simulink model "microgrid_top"  (R2025a)
settings: Solver=FixedStepDiscrete  StartTime=0.0  StopTime=86400  FixedStep=Ts  RelTol=1e-3
InitFcn:
  | init_microgrid
undefined symbols (not defined in the file): d, dt, Emax, G_clear_day, Ion, Lithium, Pmax, prof, sig, SoC_min, T_amb_day, t_day, t_hour, Tc, th1, th1_act, th2, th2_act, Ts
libraries: spsSeriesRLCBranchLib x9, spsMosfetLib x8, simulink x7, spsIGBTDiodeLib x4, slpidlib x4, spsIdealSwitchLib x4, spsVoltageMeasurementLib x4, spsParallelRLCLoadLib x3, spsPWMGeneratorDCDCLib x2, spsCurrentMeasurementLib x2, spsBatteryLib x1, spsFirstOrderFilterLib x1
settings Model: Creator=mdnih  LastModifiedBy=mdnih
settings SolverCC: AutoInsertRateTranBlk=on

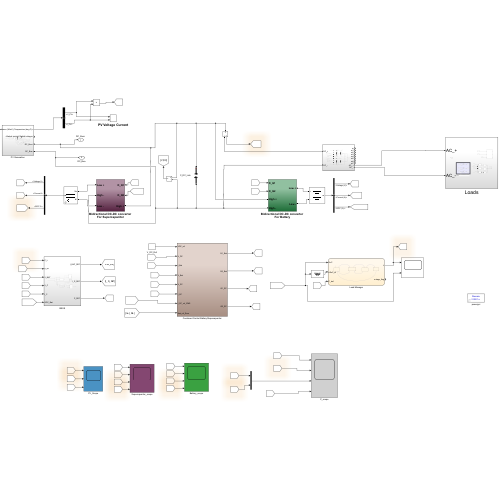
[thumbnail: Simulink's stored preview of the top-level diagram]
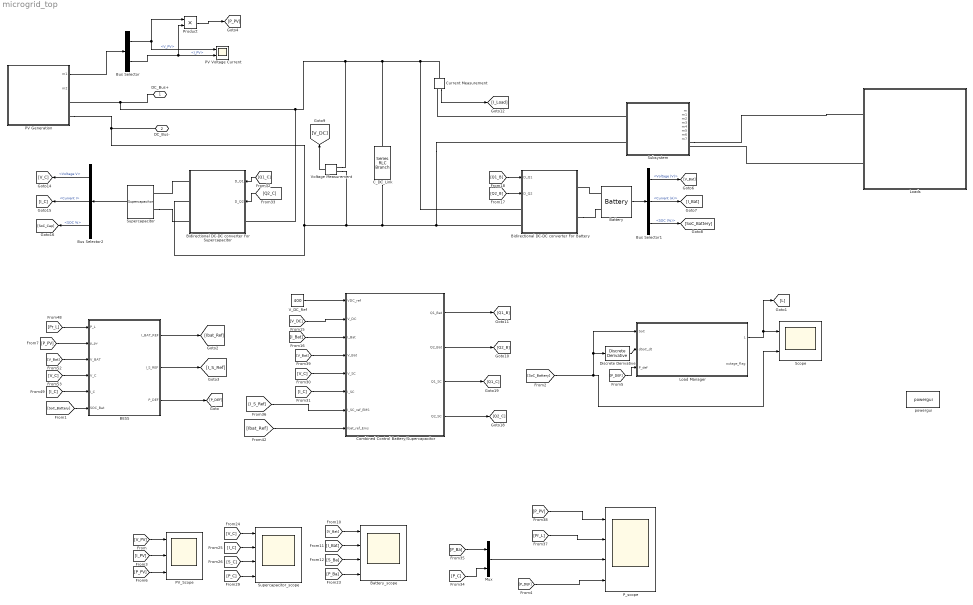
== system microgrid_top ==
  BESS : Subsystem
  Battery : spsBatteryLib/Battery  BatType=Lithium-Ion  NomV=24  NomQ=14  SOC=50  Batt_Tr=0.1  PresetModel=on  MaxQ=14  MinV=18  FullV=27.9357  Dis_rate=6.087  R=0.017143  Normal_OP=12.6609  expZone="[25.9293     0.687826]"
      settings: LibrarySourceBlock=electricdrivelib/Extra Sources/Battery
  "Battery_scope " : Scope  NumInputPorts=4
      settings: ActiveDisplayYMinimum=-3.2401785596786041  ActiveDisplayYMaximum=29.161607037107444  DataLoggingVariableName=ScopeData2
  Bidirectional DC-DC converter For Battery : Subsystem
  Bidirectional DC-DC converter For Supercapacitor : Subsystem
  Bus Selector : BusSelector  OutputSignals=V_PV,I_PV
  Bus Selector1 : BusSelector  OutputSignals=Voltage (V),Current (A),SOC (%)
  Bus Selector2 : BusSelector  OutputSignals=Voltage V,Current I,SOC %
  C_DC_Link : spsSeriesRLCBranchLib/Series RLC Branch  LConnTagsString=__new0  RConnTagsString=__new0  BranchType=C  Resistance=1  Inductance=1e-3  SetiL0=off  InitialCurrent=0  Capacitance=300e-6  Setx0=off  InitialVoltage=0  Measurements=None
  Combined Control Battery/Supercapacitor : Subsystem
  Current Measurement : spsCurrentMeasurementLib/Current Measurement  PhasorSimulation=off  OutputType=Complex  PSBequivalent=0
  Discrete Derivative : simulink/Discrete/Discrete Derivative  gainval=1.0  ICPrevScaledInput=0.0  OutMin=[]  OutMax=[]  OutDataType=fixdt(1, 16)  OutScaling=2^-10  DoSatur=off
  Load Manager : Stateflow chart  TreatAsAtomicUnit=on
  Loads : Subsystem
  Mux : Mux  Inputs=2
  PV Generation : Subsystem
  PV Voltage Current : Scope  NumInputPorts=2
  PV_Scope : Scope  NumInputPorts=3
      settings: ActiveDisplayYMinimum=-5.01178  ActiveDisplayYMaximum=45.10602  DataLoggingVariableName=ScopeData3
  P_scope : Scope  NumInputPorts=4
      settings: ActiveDisplayYMinimum=-1  ActiveDisplayYMaximum=1  DataLoggingVariableName=ScopeData4
  Product : Product
  Scope : Scope  NumInputPorts=2
      settings: ActiveDisplayYMinimum=-0.24999999999999994  ActiveDisplayYMaximum=2.25
  Subsystem : Subsystem
  Supercapacitor : spsSupercapacitorLib/Supercapacitor  C=29  Rdc=0.003  Voltage=32  Ns=1  Np=1  Vinit=32  Temp=25  Nc=1  r=1e-9  epsilon=6.0208e-10  Ioc=10  Vself="[48  47.8  47.06  44.65]"
      settings: LibrarySourceBlock=electricdrivelib/Extra Sources/Supercapacitor
  Supercapacitor_scope : Scope  NumInputPorts=4
      settings: ActiveDisplayYMinimum=31.852425698954992  ActiveDisplayYMaximum=32.0163550827263  DataLoggingVariableName=ScopeData5
  V_DC_Ref : Constant  Value=400
  Voltage Measurement : spsVoltageMeasurementLib/Voltage Measurement  PhasorSimulation=off  OutputType=Complex  PSBequivalent=0
  powergui : sps_lib/powergui  Priority=1  SimulationMode=Discrete  SampleTime=Ts  frequency=60  Iterations=50  frequencyindice=0  Pbase=100e6  ErrMax=1e-4  UnitsV=kV  UnitsW=MW  buscounter=0  FunctionMessages=off  echomessages=off  EnableUseOfTLC=off  CurrentSourceSwitches=off  DisableSnubberDevices=off  DisableRonSwitches=off  DisableVfSwitches=off  DisplayEquations=off  AutomaticDiscreteSolvers=off  SolverType=Tustin/Backward Euler (TBE)  Interpol=off  ExternalGateDelay=off  methode=off  Ts=100  x0status=blocks  SPID=on  SwTol=0  HookPort=off  NonlinearTolerance=1e-4  nMaxIteration=100  ContinueOnMaxIteration=off  RestoreLinks=warning  ResistiveCurrentMeasurement=off  Frange=[0:2:500]  Ylog=off  Xlog=on  ShowGrid=off  save=off  variable=ZData  structure=0  ZoomFFT=off  StartTime=0.0  cycles=1  DisplayStyle=1  fundamental=60  FreqAxis=off  MaxFrequency=1000  frequencyindicesteady=1  RmsSteady=1  display=off
  DC_Bus+ : PMIOPort  Side=Right
  DC_Bus- : PMIOPort  Port=2  Side=Left
  wires:
  [Q1_B] -> Bidirectional DC-DC converter For Battery/1(D_Q1)
  Bus Selector2/1 -> [V_C]  "<Voltage V>"
  [Q2_B] -> Bidirectional DC-DC converter For Battery/2(D_Q2)
  Battery/1 -> Bus Selector1/1
  Bus Selector1/3 -> [SoC_Battery]  "<SOC (%)>"
  Bus Selector1/2 -> [I_Bat]  "<Current (A)>"
  Voltage Measurement/1 -> [V_DC]
  Bus Selector1/1 -> [V_Bat]  "<Voltage (V)>"
  [Q2_C] -> Bidirectional DC-DC converter For Supercapacitor/2(D_Q2)
  Bus Selector2/2 -> [I_C]  "<Current I>"
  Supercapacitor/1 -> Bus Selector2/1
  Current Measurement/1 -> [I_Load]
  Bus Selector2/3 -> [SoC_Cap]  "<SOC %>"
  [Q1_C] -> Bidirectional DC-DC converter For Supercapacitor/1(D_Q1)
  [SoC_Battery] -> BESS/6(SOC_Bat)
  [Pr_L] -> BESS/1(P_L)
  [V_C] -> BESS/4(V_C)
  [P_PV] -> BESS/2(p_pv)
  [V_Bat] -> BESS/3(V_BAT)
  BESS/2(I_S_REF) -> [I_S_Ref]
  BESS/3(P_DEF) -> [P_DEF]
  BESS/1(I_BAT_REF) -> [Ibat_Ref]
  [I_C] -> BESS/5(I_C)
  [SoC_Battery] -> Scope/2, Discrete Derivative/1, Load Manager/1(SoC)
  PV Generation/1(m1) -> Bus Selector/1
  Bus Selector/1 -> Product/1, PV Voltage Current/1  "<V_PV>"
  Bus Selector/2 -> Product/2, PV Voltage Current/2  "<I_PV>"
  [I_S_Ref] -> Combined Control Battery/Supercapacitor/7(I_SC_ref_EMS)
  [V_Bat] -> Combined Control Battery/Supercapacitor/4(V_Bat)
  Combined Control Battery/Supercapacitor/3(Q1_SC) -> [Q1_C]
  Combined Control Battery/Supercapacitor/4(Q2_SC) -> [Q2_C]
  [V_C] -> Combined Control Battery/Supercapacitor/5("V_SC ")
  Combined Control Battery/Supercapacitor/2(Q2_Bat) -> [Q2_B]
  [I_Bat] -> Combined Control Battery/Supercapacitor/3(I_Bat)
  Combined Control Battery/Supercapacitor/1(Q1_Bat) -> [Q1_B]
  [I_C] -> Combined Control Battery/Supercapacitor/6(I_SC)
  [Ibat_Ref] -> Combined Control Battery/Supercapacitor/8(Ibat_ref_Ems)
  [V_DC] -> Combined Control Battery/Supercapacitor/2(V_DC)
  V_DC_Ref/1 -> Combined Control Battery/Supercapacitor/1(VDC_ref)
  [P_Ba] -> "Battery_scope "/4
  [P_Ba] -> Mux/1
  [Pr_L] -> P_scope/2
  [V_PV] -> PV_Scope/1
  [P_C] -> Mux/2
  [P_DEF] -> P_scope/4
  [S_C] -> Supercapacitor_scope/3
  [V_C] -> Supercapacitor_scope/1
  [I_Bat] -> "Battery_scope "/2
  [P_PV] -> P_scope/1
  [P_PV] -> PV_Scope/3
  [S_Ba] -> "Battery_scope "/3
  Mux/1 -> P_scope/3
  [P_C] -> Supercapacitor_scope/4
  [V_Bat] -> "Battery_scope "/1
  [I_C] -> Supercapacitor_scope/2
  [I_PV] -> PV_Scope/2
  Load Manager/1(L) -> [L], Scope/1
  Discrete Derivative/1 -> Load Manager/2(dSoC_dt)
  [P_DEF] -> Load Manager/3(P_def)
  Product/1 -> [P_PV]
  connections:
  PV Generation/RConn2 -- DC_Bus-/RConn1 -- Voltage Measurement/LConn2 -- Subsystem/LConn2 -- Bidirectional DC-DC converter For Battery/LConn2 -- C_DC_Link/RConn1 -- Bidirectional DC-DC converter For Supercapacitor/RConn2
  DC_Bus+/RConn1 -- PV Generation/RConn1 -- Voltage Measurement/LConn1 -- Current Measurement/LConn1 -- Bidirectional DC-DC converter For Battery/LConn1 -- C_DC_Link/LConn1 -- Bidirectional DC-DC converter For Supercapacitor/LConn1
  Subsystem/LConn1 -- Current Measurement/RConn1
  Supercapacitor/LConn2 -- Bidirectional DC-DC converter For Supercapacitor/RConn3
  Bidirectional DC-DC converter For Supercapacitor/RConn1 -- Supercapacitor/LConn1
  Battery/LConn1 -- Bidirectional DC-DC converter For Battery/RConn1
  Bidirectional DC-DC converter For Battery/RConn2 -- Battery/LConn2
  Subsystem/RConn1 -- Loads/LConn1
  Loads/LConn2 -- Subsystem/RConn2

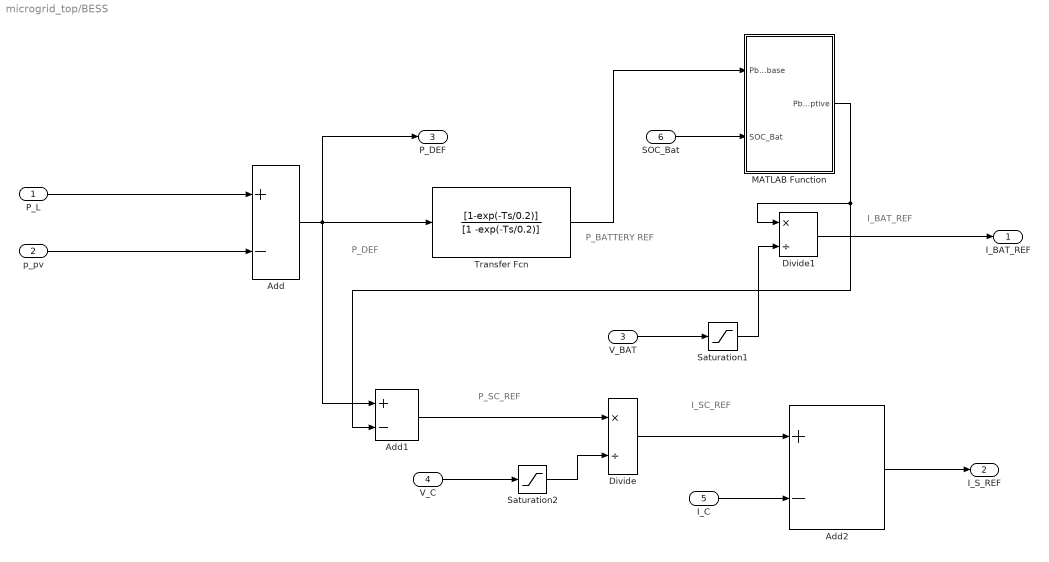
== system microgrid_top/BESS ==
  note: P_SC_REF
  note: I_BAT_REF
  note: P_DEF
  note: P_BATTERY REF
  note: I_SC_REF
  P_L : Inport
  p_pv : Inport  Port=2
  V_BAT : Inport  Port=3
  V_C : Inport  Port=4
  I_C : Inport  Port=5
  SOC_Bat : Inport  Port=6
  Add : Sum  Inputs=+-
  Add1 : Sum  Inputs=+-
  Add2 : Sum  Inputs=+-
  Divide : Product  Inputs=*/
  Divide1 : Product  Inputs=*/
  MATLAB Function : MATLAB Function  TreatAsAtomicUnit=on
  Saturation1 : Saturate  UpperLimit=1000  LowerLimit=1
  Saturation2 : Saturate  UpperLimit=1000  LowerLimit=1
  Transfer Fcn : DiscreteTransferFcn  Numerator=[1-exp(-Ts/0.2)]  Denominator=[1 -exp(-Ts/0.2)]  SampleTime=Ts
  I_BAT_REF : Outport
  I_S_REF : Outport  Port=2
  P_DEF : Outport  Port=3
  wires:
  Transfer Fcn/1 -> MATLAB Function/1(Pbat_base)
  Add1/1 -> Divide/1
  Saturation2/1 -> Divide/2
  MATLAB Function/1(Pbat_adaptive) -> Add1/2, Divide1/1
  Add/1 -> P_DEF/1, Transfer Fcn/1, Add1/1
  Saturation1/1 -> Divide1/2
  Divide/1 -> Add2/1
  P_L/1 -> Add/1
  p_pv/1 -> Add/2
  SOC_Bat/1 -> MATLAB Function/2(SOC_Bat)
  Divide1/1 -> I_BAT_REF/1
  Add2/1 -> I_S_REF/1
  V_BAT/1 -> Saturation1/1
  I_C/1 -> Add2/2
  V_C/1 -> Saturation2/1

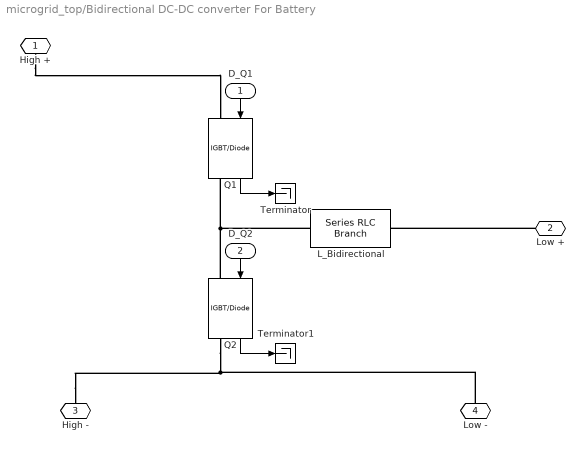
== system microgrid_top/Bidirectional DC-DC converter For Battery ==
  D_Q1 : Inport
  D_Q2 : Inport  Port=2
  L_Bidirectional : spsSeriesRLCBranchLib/Series RLC Branch  LConnTagsString=__new0  RConnTagsString=__new0  BranchType=RL  Resistance=0.05  Inductance=0.3e-3  SetiL0=off  InitialCurrent=0  Capacitance=1e-6  Setx0=off  InitialVoltage=0  Measurements=None
  Q1 : spsIGBTDiodeLib/IGBT//Diode  Ron=1e-3  Rs=1e5  Cs=inf  Measurements=on
  Q2 : spsIGBTDiodeLib/IGBT//Diode  Ron=1e-3  Rs=1e5  Cs=inf  Measurements=on
  Terminator : Terminator
  Terminator1 : Terminator
  High + : PMIOPort  Side=Left
  Low + : PMIOPort  Port=2  Side=Right
  High - : PMIOPort  Port=3  Side=Left
  Low - : PMIOPort  Port=4  Side=Right
  wires:
  D_Q2/1 -> Q2/1
  D_Q1/1 -> Q1/1
  Q1/1 -> Terminator/1
  Q2/1 -> Terminator1/1
  connections:
  High -/RConn1 -- Low -/RConn1 -- Q2/RConn1
  High +/RConn1 -- Q1/LConn1
  Low +/RConn1 -- L_Bidirectional/RConn1
  Q2/LConn1 -- L_Bidirectional/LConn1 -- Q1/RConn1

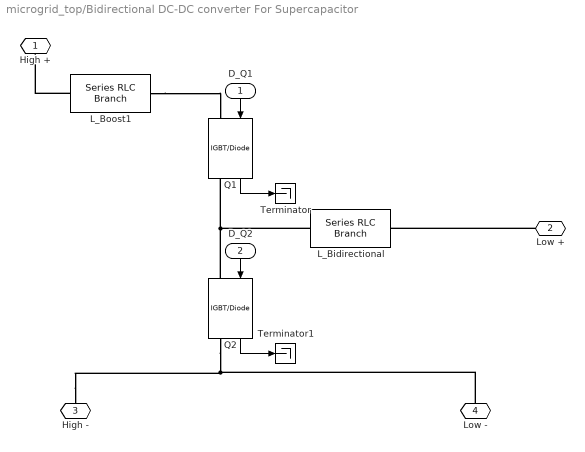
== system microgrid_top/Bidirectional DC-DC converter For Supercapacitor ==
  D_Q1 : Inport
  D_Q2 : Inport  Port=2
  L_Bidirectional : spsSeriesRLCBranchLib/Series RLC Branch  LConnTagsString=__new0  RConnTagsString=__new0  BranchType=RL  Resistance=0.05  Inductance=0.355e-3  SetiL0=off  InitialCurrent=0  Capacitance=1e-6  Setx0=off  InitialVoltage=0  Measurements=None
  L_Boost1 : spsSeriesRLCBranchLib/Series RLC Branch  LConnTagsString=__new0  RConnTagsString=__new0  BranchType=L  Resistance=0.05  Inductance=1.5e-3  SetiL0=off  InitialCurrent=0  Capacitance=1e-6  Setx0=off  InitialVoltage=0  Measurements=None
  Q1 : spsIGBTDiodeLib/IGBT//Diode  Ron=1e-3  Rs=1e5  Cs=inf  Measurements=on
  Q2 : spsIGBTDiodeLib/IGBT//Diode  Ron=1e-3  Rs=1e5  Cs=inf  Measurements=on
  Terminator : Terminator
  Terminator1 : Terminator
  High + : PMIOPort  Side=Left
  Low + : PMIOPort  Port=2  Side=Right
  High - : PMIOPort  Port=3  Side=Right
  Low - : PMIOPort  Port=4  Side=Right
  wires:
  D_Q2/1 -> Q2/1
  D_Q1/1 -> Q1/1
  Q1/1 -> Terminator/1
  Q2/1 -> Terminator1/1
  connections:
  High -/RConn1 -- Low -/RConn1 -- Q2/RConn1
  Low +/RConn1 -- L_Bidirectional/RConn1
  Q2/LConn1 -- L_Bidirectional/LConn1 -- Q1/RConn1
  L_Boost1/RConn1 -- Q1/LConn1
  L_Boost1/LConn1 -- High +/RConn1

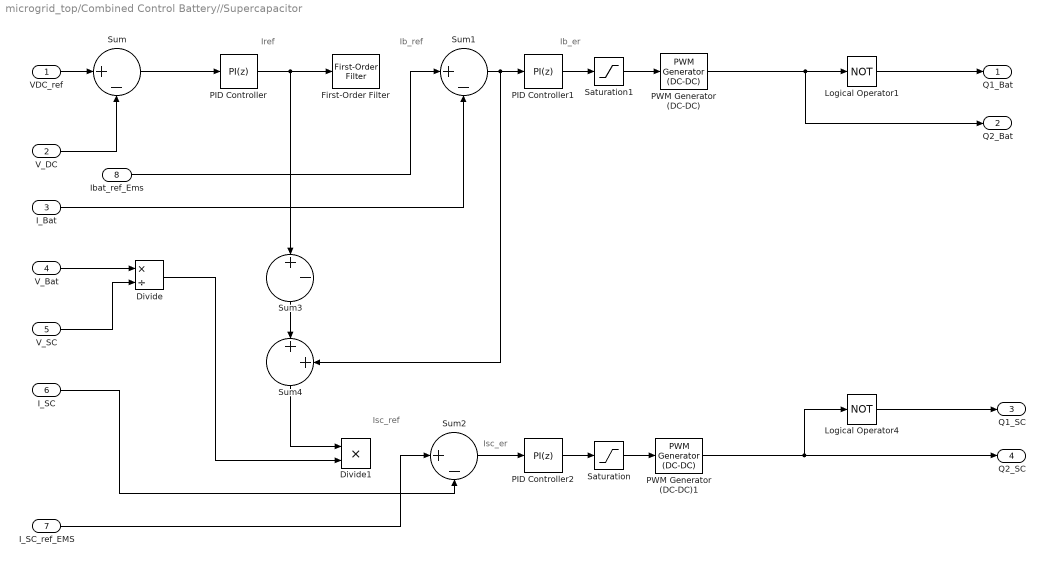
== system microgrid_top/Combined Control Battery//Supercapacitor ==
  note: Isc_er
  note: Isc_ref
  note: Ib_er
  note: Ib_ref
  note: Iref
  VDC_ref : Inport
  V_DC : Inport  Port=2
  I_Bat : Inport  Port=3
  V_Bat : Inport  Port=4
  "V_SC " : Inport  Port=5
  I_SC : Inport  Port=6
  I_SC_ref_EMS : Inport  Port=7
  Ibat_ref_Ems : Inport  Port=8
  Divide : Product  Inputs=*/
  Divide1 : Product  Inputs=**
  First-Order Filter : spsFirstOrderFilterLib/First-Order Filter  FilterType=Lowpass  Tc=0.015  Ts=Ts  Initialize=off  Vac_Init=[0, 0, 60]  Vdc_Init=0  PlotResponse=off  FreqRange="[0,  200,  1]"
  Logical Operator1 : Logic  Operator=NOT  AllPortsSameDT=off  OutDataTypeStr=boolean
  Logical Operator4 : Logic  Operator=NOT  AllPortsSameDT=off  OutDataTypeStr=boolean
  PID Controller : slpidlib/PID Controller  Controller=PI  Form=Parallel  TimeDomain=Discrete-time  UseExternalTs=off  SampleTime=Ts  IntegratorMethod=Backward Euler  FilterMethod=Backward Euler  ControllerParametersSource=internal  P=1.477  I=3077  UseKiTs=off  D=0  UseExternalDerivativeSource=off  N=100  UseFilter=on  TunerSelectOption=Transfer Function Based (PID Tuner App)  InitialConditionSource=internal  InitialConditionForIntegrator=0  InitialConditionForFilter=0  DifferentiatorICPrevScaledInput=0  ExternalReset=none  TrackingMode=off  Kt=1  LimitOutput=off  SatLimitsSource=internal  UpperSaturationLimit=inf  LowerSaturationLimit=-inf  LinearizeAsGain=on  AntiWindupMode=none  Kb=1  LimitIntegrator=off  UpperIntegratorSaturationLimit=inf  LowerIntegratorSaturationLimit=-inf  POutMin=[]  POutMax=[]  IOutMin=[]  IOutMax=[]  DOutMin=[]  DOutMax=[]  NOutMin=[]  NOutMax=[]  SumOutMin=[]  SumOutMax=[]  SaturationOutMin=[]  SaturationOutMax=[]  PParamMin=[]  PParamMax=[]  IParamMin=[]  IParamMax=[]  DParamMin=[]  DParamMax=[]  NParamMin=[]  NParamMax=[]  KbParamMin=[]  KbParamMax=[]  KtParamMin=[]  KtParamMax=[]  KbOutMin=[]  KbOutMax=[]  KtOutMin=[]  KtOutMax=[]  IntegratorOutMin=[]  IntegratorOutMax=[]  FilterOutMin=[]  FilterOutMax=[]  SumI1OutMin=[]  SumI1OutMax=[]  SumI2OutMin=[]  SumI2OutMax=[]  SumI3OutMin=[]  SumI3OutMax=[]  SumI4OutMin=[]  SumI4OutMax=[]  SumDOutMin=[]  SumDOutMax=[]  DifferentiatorOutMin=[]  DifferentiatorOutMax=[]  FilterDiffOutCoefMin=[]  FilterDiffOutCoefMax=[]  ReciprocalOutMin=[]  ReciprocalOutMax=[]  SumDenOutMin=[]  SumDenOutMax=[]  SumNumOutMin=[]  SumNumOutMax=[]  DivideOutMin=[]  DivideOutMax=[]  UdiffTsProdOutMin=[]  UdiffTsProdOutMax=[]  NTsProdOutMin=[]  NTsProdOutMax=[]  UintegralTsProdOutMin=[]  UintegralTsProdOutMax=[]  UngainTsProdOutMin=[]  UngainTsProdOutMax=[]  ClampingZeroOutDataTypeStr=Inherit: Inherit via back propagation  ClampingZeroOutMin=[]  ClampingZeroOutMax=[]  FilterDenConstantOutDataTypeStr=Inherit: Inherit via back propagation  FilterDenConstantOutMin=[]  FilterDenConstantOutMax=[]  PCopyOutDataTypeStr=Inherit: Inherit via back propagation  PCopyOutMin=[]  PCopyOutMax=[]  NCopyOutDataTypeStr=Inherit: Inherit via back propagation  NCopyOutMin=[]  NCopyOutMax=[]  IntegratorContinuousStateAttributes=''  IntegratorStateMustResolveToSignalObject=off  IntegratorRTWStateStorageClass=Auto  FilterContinuousStateAttributes=''  FilterStateMustResolveToSignalObject=off  FilterRTWStateStorageClass=Auto  ParallelPVariant=InternalParameters  IdealPVariant=Disabled  IVariant=InternalParameters  DVariant=Disabled  IntegratorVariant=Discrete  SatVariant=Disabled  AWVariant=Passthrough  PCopyVariant=Disabled  TRVariant=Disabled  FdbkBlocksVariant=Forward  IdealPFdbkVariant=Disabled  SatFdbkVariant=Disabled  DerivativeFilterVariant=Disabled  NVariant=Disabled  NCopyVariant=Disabled_SignalSpec  FilterICVariant=Disabled  IntegratorICVariant=InternalICs  ExternalResetVariant=Disabled  TRSumVariant=Passthrough  SumFdbkVariant=Disabled  SumVariant=Sum_PI  TsampFilterVariant=InternalTs  TsampNgainVariant=Passthrough  TsampIntegralVariant=Disabled_SignalSpec  ExternalSaturationOutDataTypeStr=Inherit: Same as second input  DerivativeSourceVariant=Disabled  PreIntVariant=InternalPreInt
  PID Controller1 : slpidlib/PID Controller  Controller=PI  Form=Parallel  TimeDomain=Discrete-time  UseExternalTs=off  SampleTime=Ts  IntegratorMethod=Backward Euler  FilterMethod=Backward Euler  ControllerParametersSource=internal  P=0.043  I=0.65  UseKiTs=off  D=0  UseExternalDerivativeSource=off  N=100  UseFilter=on  TunerSelectOption=Transfer Function Based (PID Tuner App)  InitialConditionSource=internal  InitialConditionForIntegrator=0  InitialConditionForFilter=0  DifferentiatorICPrevScaledInput=0  ExternalReset=none  TrackingMode=off  Kt=1  LimitOutput=off  SatLimitsSource=internal  UpperSaturationLimit=inf  LowerSaturationLimit=-inf  LinearizeAsGain=on  AntiWindupMode=none  Kb=1  LimitIntegrator=off  UpperIntegratorSaturationLimit=inf  LowerIntegratorSaturationLimit=-inf  POutMin=[]  POutMax=[]  IOutMin=[]  IOutMax=[]  DOutMin=[]  DOutMax=[]  NOutMin=[]  NOutMax=[]  SumOutMin=[]  SumOutMax=[]  SaturationOutMin=[]  SaturationOutMax=[]  PParamMin=[]  PParamMax=[]  IParamMin=[]  IParamMax=[]  DParamMin=[]  DParamMax=[]  NParamMin=[]  NParamMax=[]  KbParamMin=[]  KbParamMax=[]  KtParamMin=[]  KtParamMax=[]  KbOutMin=[]  KbOutMax=[]  KtOutMin=[]  KtOutMax=[]  IntegratorOutMin=[]  IntegratorOutMax=[]  FilterOutMin=[]  FilterOutMax=[]  SumI1OutMin=[]  SumI1OutMax=[]  SumI2OutMin=[]  SumI2OutMax=[]  SumI3OutMin=[]  SumI3OutMax=[]  SumI4OutMin=[]  SumI4OutMax=[]  SumDOutMin=[]  SumDOutMax=[]  DifferentiatorOutMin=[]  DifferentiatorOutMax=[]  FilterDiffOutCoefMin=[]  FilterDiffOutCoefMax=[]  ReciprocalOutMin=[]  ReciprocalOutMax=[]  SumDenOutMin=[]  SumDenOutMax=[]  SumNumOutMin=[]  SumNumOutMax=[]  DivideOutMin=[]  DivideOutMax=[]  UdiffTsProdOutMin=[]  UdiffTsProdOutMax=[]  NTsProdOutMin=[]  NTsProdOutMax=[]  UintegralTsProdOutMin=[]  UintegralTsProdOutMax=[]  UngainTsProdOutMin=[]  UngainTsProdOutMax=[]  ClampingZeroOutDataTypeStr=Inherit: Inherit via back propagation  ClampingZeroOutMin=[]  ClampingZeroOutMax=[]  FilterDenConstantOutDataTypeStr=Inherit: Inherit via back propagation  FilterDenConstantOutMin=[]  FilterDenConstantOutMax=[]  PCopyOutDataTypeStr=Inherit: Inherit via back propagation  PCopyOutMin=[]  PCopyOutMax=[]  NCopyOutDataTypeStr=Inherit: Inherit via back propagation  NCopyOutMin=[]  NCopyOutMax=[]  IntegratorContinuousStateAttributes=''  IntegratorStateMustResolveToSignalObject=off  IntegratorRTWStateStorageClass=Auto  FilterContinuousStateAttributes=''  FilterStateMustResolveToSignalObject=off  FilterRTWStateStorageClass=Auto  ParallelPVariant=InternalParameters  IdealPVariant=Disabled  IVariant=InternalParameters  DVariant=Disabled  IntegratorVariant=Discrete  SatVariant=Disabled  AWVariant=Passthrough  PCopyVariant=Disabled  TRVariant=Disabled  FdbkBlocksVariant=Forward  IdealPFdbkVariant=Disabled  SatFdbkVariant=Disabled  DerivativeFilterVariant=Disabled  NVariant=Disabled  NCopyVariant=Disabled_SignalSpec  FilterICVariant=Disabled  IntegratorICVariant=InternalICs  ExternalResetVariant=Disabled  TRSumVariant=Passthrough  SumFdbkVariant=Disabled  SumVariant=Sum_PI  TsampFilterVariant=InternalTs  TsampNgainVariant=Passthrough  TsampIntegralVariant=Disabled_SignalSpec  ExternalSaturationOutDataTypeStr=Inherit: Same as second input  DerivativeSourceVariant=Disabled  PreIntVariant=InternalPreInt
  PID Controller2 : slpidlib/PID Controller  Controller=PI  Form=Parallel  TimeDomain=Discrete-time  UseExternalTs=off  SampleTime=Ts  IntegratorMethod=Backward Euler  FilterMethod=Backward Euler  ControllerParametersSource=internal  P=0.45  I=14800  UseKiTs=off  D=0  UseExternalDerivativeSource=off  N=100  UseFilter=on  TunerSelectOption=Transfer Function Based (PID Tuner App)  InitialConditionSource=internal  InitialConditionForIntegrator=0  InitialConditionForFilter=0  DifferentiatorICPrevScaledInput=0  ExternalReset=none  TrackingMode=off  Kt=1  LimitOutput=off  SatLimitsSource=internal  UpperSaturationLimit=inf  LowerSaturationLimit=-inf  LinearizeAsGain=on  AntiWindupMode=none  Kb=1  LimitIntegrator=off  UpperIntegratorSaturationLimit=inf  LowerIntegratorSaturationLimit=-inf  POutMin=[]  POutMax=[]  IOutMin=[]  IOutMax=[]  DOutMin=[]  DOutMax=[]  NOutMin=[]  NOutMax=[]  SumOutMin=[]  SumOutMax=[]  SaturationOutMin=[]  SaturationOutMax=[]  PParamMin=[]  PParamMax=[]  IParamMin=[]  IParamMax=[]  DParamMin=[]  DParamMax=[]  NParamMin=[]  NParamMax=[]  KbParamMin=[]  KbParamMax=[]  KtParamMin=[]  KtParamMax=[]  KbOutMin=[]  KbOutMax=[]  KtOutMin=[]  KtOutMax=[]  IntegratorOutMin=[]  IntegratorOutMax=[]  FilterOutMin=[]  FilterOutMax=[]  SumI1OutMin=[]  SumI1OutMax=[]  SumI2OutMin=[]  SumI2OutMax=[]  SumI3OutMin=[]  SumI3OutMax=[]  SumI4OutMin=[]  SumI4OutMax=[]  SumDOutMin=[]  SumDOutMax=[]  DifferentiatorOutMin=[]  DifferentiatorOutMax=[]  FilterDiffOutCoefMin=[]  FilterDiffOutCoefMax=[]  ReciprocalOutMin=[]  ReciprocalOutMax=[]  SumDenOutMin=[]  SumDenOutMax=[]  SumNumOutMin=[]  SumNumOutMax=[]  DivideOutMin=[]  DivideOutMax=[]  UdiffTsProdOutMin=[]  UdiffTsProdOutMax=[]  NTsProdOutMin=[]  NTsProdOutMax=[]  UintegralTsProdOutMin=[]  UintegralTsProdOutMax=[]  UngainTsProdOutMin=[]  UngainTsProdOutMax=[]  ClampingZeroOutDataTypeStr=Inherit: Inherit via back propagation  ClampingZeroOutMin=[]  ClampingZeroOutMax=[]  FilterDenConstantOutDataTypeStr=Inherit: Inherit via back propagation  FilterDenConstantOutMin=[]  FilterDenConstantOutMax=[]  PCopyOutDataTypeStr=Inherit: Inherit via back propagation  PCopyOutMin=[]  PCopyOutMax=[]  NCopyOutDataTypeStr=Inherit: Inherit via back propagation  NCopyOutMin=[]  NCopyOutMax=[]  IntegratorContinuousStateAttributes=''  IntegratorStateMustResolveToSignalObject=off  IntegratorRTWStateStorageClass=Auto  FilterContinuousStateAttributes=''  FilterStateMustResolveToSignalObject=off  FilterRTWStateStorageClass=Auto  ParallelPVariant=InternalParameters  IdealPVariant=Disabled  IVariant=InternalParameters  DVariant=Disabled  IntegratorVariant=Discrete  SatVariant=Disabled  AWVariant=Passthrough  PCopyVariant=Disabled  TRVariant=Disabled  FdbkBlocksVariant=Forward  IdealPFdbkVariant=Disabled  SatFdbkVariant=Disabled  DerivativeFilterVariant=Disabled  NVariant=Disabled  NCopyVariant=Disabled_SignalSpec  FilterICVariant=Disabled  IntegratorICVariant=InternalICs  ExternalResetVariant=Disabled  TRSumVariant=Passthrough  SumFdbkVariant=Disabled  SumVariant=Sum_PI  TsampFilterVariant=InternalTs  TsampNgainVariant=Passthrough  TsampIntegralVariant=Disabled_SignalSpec  ExternalSaturationOutDataTypeStr=Inherit: Same as second input  DerivativeSourceVariant=Disabled  PreIntVariant=InternalPreInt
  PWM Generator (DC-DC) : spsPWMGeneratorDCDCLib/PWM Generator (DC-DC)  Fsw=16000  Ts=Ts
  PWM Generator (DC-DC)1 : spsPWMGeneratorDCDCLib/PWM Generator (DC-DC)  Fsw=16000  Ts=Ts
  Saturation : Saturate  UpperLimit=1  LowerLimit=0
  Saturation1 : Saturate  UpperLimit=1  LowerLimit=0
  Sum{,1..3} (4 alike) : Sum  Inputs=|+-
  Sum4 : Sum  Inputs=|++
  Q1_Bat : Outport
  Q2_Bat : Outport  Port=2
  Q1_SC : Outport  Port=3
  Q2_SC : Outport  Port=4
  wires:
  Sum1/1 -> PID Controller1/1, Sum4/2
  PWM Generator (DC-DC)/1 -> Logical Operator1/1, Q2_Bat/1
  I_Bat/1 -> Sum1/2
  I_SC/1 -> Sum2/2
  Sum2/1 -> PID Controller2/1
  Logical Operator1/1 -> Q1_Bat/1
  Sum/1 -> PID Controller/1
  VDC_ref/1 -> Sum/1
  V_DC/1 -> Sum/2
  V_Bat/1 -> Divide/1
  "V_SC "/1 -> Divide/2
  Logical Operator4/1 -> Q1_SC/1
  PWM Generator (DC-DC)1/1 -> Q2_SC/1, Logical Operator4/1
  PID Controller/1 -> First-Order Filter/1, Sum3/1
  Sum3/1 -> Sum4/1
  Divide/1 -> Divide1/2
  Sum4/1 -> Divide1/1
  PID Controller2/1 -> Saturation/1
  Saturation/1 -> PWM Generator (DC-DC)1/1
  PID Controller1/1 -> Saturation1/1
  Saturation1/1 -> PWM Generator (DC-DC)/1
  I_SC_ref_EMS/1 -> Sum2/1
  Ibat_ref_Ems/1 -> Sum1/1

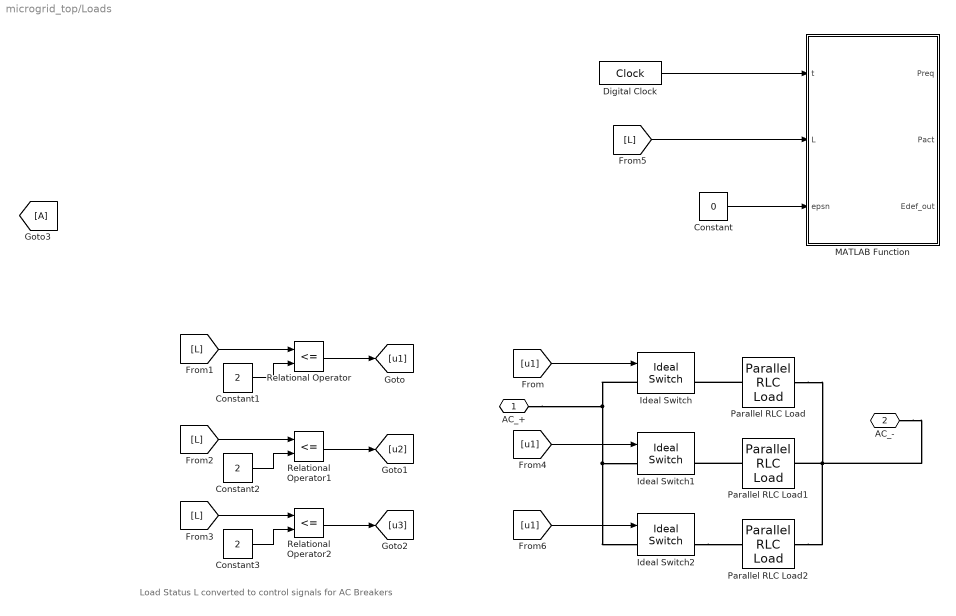
== system microgrid_top/Loads ==
  note: Load Status L converted to control signals
      | for AC Breakers
  Constant : Constant  Value=0
  Constant1 : Constant  Value=2
  Constant2 : Constant  Value=2
  Constant3 : Constant  Value=2
  Digital Clock : DigitalClock  SampleTime=dt
  Goto3 : Goto
  Ideal Switch : spsIdealSwitchLib/Ideal Switch  Ron=0.001  Lon=0  IC=0  Rs=1e5  Cs=inf  Measurements=on
  Ideal Switch1 : spsIdealSwitchLib/Ideal Switch  Ron=0.001  Lon=0  IC=0  Rs=1e5  Cs=inf  Measurements=on
  Ideal Switch2 : spsIdealSwitchLib/Ideal Switch  Ron=0.001  Lon=0  IC=0  Rs=1e5  Cs=inf  Measurements=on
  MATLAB Function : MATLAB Function  TreatAsAtomicUnit=on
  Parallel RLC Load : spsParallelRLCLoadLib/Parallel RLC Load  LConnTagsString=a  RConnTagsString=__new0  NominalVoltage=1000  NominalFrequency=60  ActivePower=10e3  InductivePower=100  CapacitivePower=100  Setx0=off  InitialVoltage=0  SetiL0=off  InitialCurrent=0  Measurements=None  LoadType=constant Z
      settings: AttributesFormatString=\n  LibrarySourceBlock=sps_lib/Passives/Parallel RLC Load
  Parallel RLC Load1 : spsParallelRLCLoadLib/Parallel RLC Load  LConnTagsString=a  RConnTagsString=__new0  NominalVoltage=1000  NominalFrequency=60  ActivePower=10e3  InductivePower=100  CapacitivePower=100  Setx0=off  InitialVoltage=0  SetiL0=off  InitialCurrent=0  Measurements=None  LoadType=constant Z
      settings: AttributesFormatString=\n  LibrarySourceBlock=sps_lib/Passives/Parallel RLC Load
  Parallel RLC Load2 : spsParallelRLCLoadLib/Parallel RLC Load  LConnTagsString=a  RConnTagsString=__new0  NominalVoltage=1000  NominalFrequency=60  ActivePower=10e3  InductivePower=100  CapacitivePower=100  Setx0=off  InitialVoltage=0  SetiL0=off  InitialCurrent=0  Measurements=None  LoadType=constant Z
      settings: AttributesFormatString=\n  LibrarySourceBlock=sps_lib/Passives/Parallel RLC Load
  Relational Operator : RelationalOperator  Operator=<=  OutDataTypeStr=boolean  RndMeth=Simplest  InputSameDT=off
  Relational Operator1 : RelationalOperator  Operator=<=  OutDataTypeStr=boolean  RndMeth=Simplest  InputSameDT=off
  Relational Operator2 : RelationalOperator  Operator=<=  OutDataTypeStr=boolean  RndMeth=Simplest  InputSameDT=off
  AC_+ : PMIOPort  Side=Left
  AC_- : PMIOPort  Port=2  Side=Left
  wires:
  Digital Clock/1 -> MATLAB Function/1(t)
  [L] -> MATLAB Function/2(L)
  Constant/1 -> MATLAB Function/3(epsn)
  [L] -> Relational Operator/1
  Constant1/1 -> Relational Operator/2
  Constant2/1 -> Relational Operator1/2
  [L] -> Relational Operator1/1
  [L] -> Relational Operator2/1
  Constant3/1 -> Relational Operator2/2
  Relational Operator/1 -> [u1]
  Relational Operator2/1 -> [u3]
  Relational Operator1/1 -> [u2]
  [u1] -> Ideal Switch/1
  [u1] -> Ideal Switch1/1
  [u1] -> Ideal Switch2/1
  connections:
  Ideal Switch/LConn1 -- Ideal Switch2/LConn1 -- Ideal Switch1/LConn1 -- AC_+/RConn1
  Parallel RLC Load/LConn1 -- Ideal Switch/RConn1
  Parallel RLC Load1/LConn1 -- Ideal Switch1/RConn1
  Ideal Switch2/RConn1 -- Parallel RLC Load2/LConn1
  Parallel RLC Load/RConn1 -- AC_-/RConn1 -- Parallel RLC Load1/RConn1 -- Parallel RLC Load2/RConn1

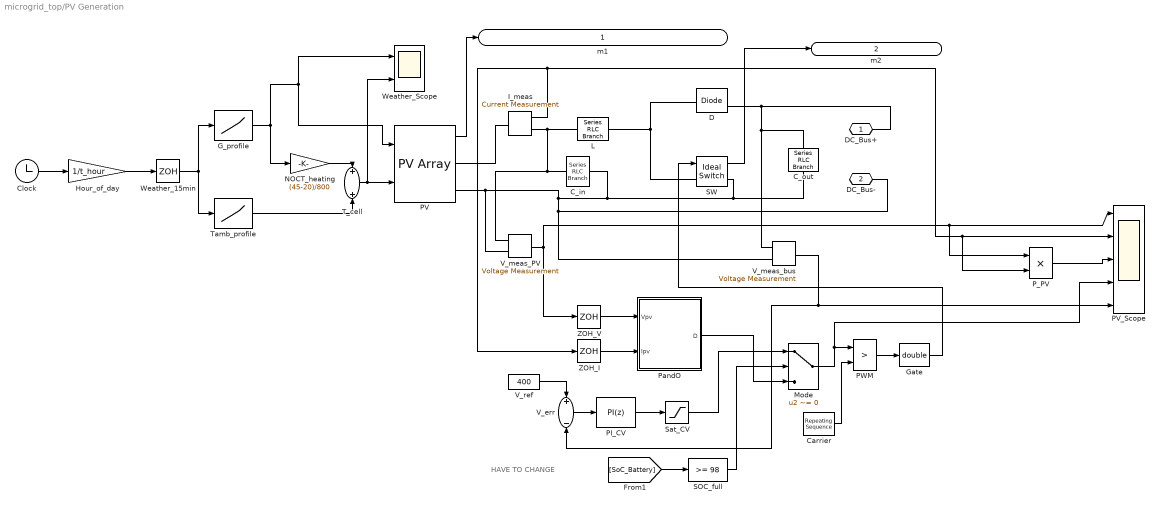
== system microgrid_top/PV Generation ==
  note: HAVE TO CHANGE
  C_in : spsSeriesRLCBranchLib/Series RLC Branch  LConnTagsString=__new0  RConnTagsString=__new0  BranchType=C  Resistance=1  Inductance=1e-3  SetiL0=off  InitialCurrent=0  Capacitance=100e-6  Setx0=off  InitialVoltage=0  Measurements=None
  C_out : spsSeriesRLCBranchLib/Series RLC Branch  LConnTagsString=__new0  RConnTagsString=__new0  BranchType=C  Resistance=1  Inductance=1e-3  SetiL0=off  InitialCurrent=0  Capacitance=100e-6  Setx0=off  InitialVoltage=0  Measurements=None
  Carrier : simulink/Sources/Repeating Sequence  rep_seq_t=[0 5e-05]  rep_seq_y=[0 1]
  Clock : Clock
  D : spsDiodeLib/Diode  Ron=0.001  Lon=0  Vf=0.8  IC=0  UseSnubber=0  Rs=500  Cs=250e-9  Measurements=on
  G_profile : Lookup_n-D  NumberOfTableDimensions=1  BreakpointsForDimension1=t_day  Table=G_clear_day  ExtrapMethod=Clip  InternalRulePriority=Speed  RndMeth=Simplest
  Gate : DataTypeConversion  OutDataTypeStr=double  SaturateOnIntegerOverflow=off  RndMeth=Floor
  Hour_of_day : Gain  Gain=1/t_hour
  I_meas : spsCurrentMeasurementLib/Current Measurement  PhasorSimulation=off  OutputType=Complex  PSBequivalent=0
  L : spsSeriesRLCBranchLib/Series RLC Branch  LConnTagsString=__new0  RConnTagsString=__new0  BranchType=L  Resistance=1  Inductance=0.8e-3  SetiL0=off  InitialCurrent=0  Capacitance=1e-6  Setx0=off  InitialVoltage=0  Measurements=None
  Mode : Switch  Criteria=u2 ~= 0  SaturateOnIntegerOverflow=off  InputSameDT=off
  NOCT_heating : Gain  Gain=(45-20)/800
  PI_CV : slpidlib/PID Controller  Controller=PI  Form=Parallel  TimeDomain=Discrete-time  UseExternalTs=off  SampleTime=0.0001  IntegratorMethod=Forward Euler  FilterMethod=Forward Euler  ControllerParametersSource=internal  P=0.001  I=0.05  UseKiTs=off  D=0  UseExternalDerivativeSource=off  N=100  UseFilter=on  TunerSelectOption=Transfer Function Based (PID Tuner App)  InitialConditionSource=internal  InitialConditionForIntegrator=0  InitialConditionForFilter=0  DifferentiatorICPrevScaledInput=0  ExternalReset=none  TrackingMode=off  Kt=1  LimitOutput=off  SatLimitsSource=internal  UpperSaturationLimit=inf  LowerSaturationLimit=-inf  LinearizeAsGain=off  AntiWindupMode=none  Kb=1  LimitIntegrator=off  UpperIntegratorSaturationLimit=inf  LowerIntegratorSaturationLimit=-inf  POutMin=[]  POutMax=[]  IOutMin=[]  IOutMax=[]  DOutMin=[]  DOutMax=[]  NOutMin=[]  NOutMax=[]  SumOutMin=[]  SumOutMax=[]  SaturationOutMin=[]  SaturationOutMax=[]  PParamMin=[]  PParamMax=[]  IParamMin=[]  IParamMax=[]  DParamMin=[]  DParamMax=[]  NParamMin=[]  NParamMax=[]  KbParamMin=[]  KbParamMax=[]  KtParamMin=[]  KtParamMax=[]  KbOutMin=[]  KbOutMax=[]  KtOutMin=[]  KtOutMax=[]  IntegratorOutMin=[]  IntegratorOutMax=[]  FilterOutMin=[]  FilterOutMax=[]  SumI1OutMin=[]  SumI1OutMax=[]  SumI2OutMin=[]  SumI2OutMax=[]  SumI3OutMin=[]  SumI3OutMax=[]  SumI4OutMin=[]  SumI4OutMax=[]  SumDOutMin=[]  SumDOutMax=[]  DifferentiatorOutMin=[]  DifferentiatorOutMax=[]  FilterDiffOutCoefMin=[]  FilterDiffOutCoefMax=[]  ReciprocalOutMin=[]  ReciprocalOutMax=[]  SumDenOutMin=[]  SumDenOutMax=[]  SumNumOutMin=[]  SumNumOutMax=[]  DivideOutMin=[]  DivideOutMax=[]  UdiffTsProdOutMin=[]  UdiffTsProdOutMax=[]  NTsProdOutMin=[]  NTsProdOutMax=[]  UintegralTsProdOutMin=[]  UintegralTsProdOutMax=[]  UngainTsProdOutMin=[]  UngainTsProdOutMax=[]  ClampingZeroOutDataTypeStr=Inherit: Inherit via back propagation  ClampingZeroOutMin=[]  ClampingZeroOutMax=[]  FilterDenConstantOutDataTypeStr=Inherit: Inherit via back propagation  FilterDenConstantOutMin=[]  FilterDenConstantOutMax=[]  PCopyOutDataTypeStr=Inherit: Inherit via back propagation  PCopyOutMin=[]  PCopyOutMax=[]  NCopyOutDataTypeStr=Inherit: Inherit via back propagation  NCopyOutMin=[]  NCopyOutMax=[]  IntegratorContinuousStateAttributes=''  IntegratorStateMustResolveToSignalObject=off  IntegratorRTWStateStorageClass=Auto  FilterContinuousStateAttributes=''  FilterStateMustResolveToSignalObject=off  FilterRTWStateStorageClass=Auto  ParallelPVariant=InternalParameters  IdealPVariant=Disabled  IVariant=InternalParameters  DVariant=Disabled  IntegratorVariant=Discrete  SatVariant=Disabled  AWVariant=Passthrough  PCopyVariant=Disabled  TRVariant=Disabled  FdbkBlocksVariant=Forward  IdealPFdbkVariant=Disabled  SatFdbkVariant=Disabled  DerivativeFilterVariant=Disabled  NVariant=Disabled  NCopyVariant=Disabled_SignalSpec  FilterICVariant=Disabled  IntegratorICVariant=InternalICs  ExternalResetVariant=Disabled  TRSumVariant=Passthrough  SumFdbkVariant=Disabled  SumVariant=Sum_PI  TsampFilterVariant=InternalTs  TsampNgainVariant=Passthrough  TsampIntegralVariant=Disabled_SignalSpec  ExternalSaturationOutDataTypeStr=Inherit: Same as second input  DerivativeSourceVariant=Disabled  PreIntVariant=InternalPreInt
      settings: LibrarySourceBlock=simulink/Discrete/Discrete PID Controller
  PV : spsPVArrayLib/PV Array  Npar=3  Nser=6  PlotType=array @ 1000 W/m2 & specified temperatures  S_vec="[ 1000  500  100 ]"  Temp_C_vec="[ 45 25  ]"  ModuleName=User-defined  PlotWhenSelected=off  Pm=400  Ncell=72  Voc=48  Isc=10.5  Vm=40  Im=10  beta_Voc_pc=-0.36099  alpha_Isc_pc=0.102  beta_Voc=-0.17328  alpha_Isc=0.01071  IL=10.576  I0=3.9433e-10  nI=1.0809  Rsh=821.7644  Rs=0.20021  RobustModel=off  RobustCellTemperature=313.3991  BAL=on  Tc=1e-6  Tfilter=5e-5
  PV_Scope : Scope  NumInputPorts=5
      settings: ActiveDisplayYMinimum=-29.860009730532969  ActiveDisplayYMaximum=268.7400875747968  DataLoggingDecimation=100  DataLoggingVariableName=pvdata
  PWM : RelationalOperator  Operator=>  OutDataTypeStr=boolean  RndMeth=Simplest  InputSameDT=off
  P_PV : Product
  PandO : MATLAB Function  TreatAsAtomicUnit=on
  SOC_full : simulink/Logic and Bit Operations/Compare To Constant  relop=>=  const=98  OutDataTypeStr=boolean
  SW : spsIdealSwitchLib/Ideal Switch  Ron=0.001  Lon=0  IC=0  Rs=1e5  Cs=inf  Measurements=on
  Sat_CV : Saturate  UpperLimit=0.85  LowerLimit=0.05
  T_cell : Sum
  Tamb_profile : Lookup_n-D  NumberOfTableDimensions=1  BreakpointsForDimension1=t_day  Table=T_amb_day  ExtrapMethod=Clip  InternalRulePriority=Speed  RndMeth=Simplest
  V_err : Sum  Inputs=+-
  V_meas_PV : spsVoltageMeasurementLib/Voltage Measurement  PhasorSimulation=off  OutputType=Complex  PSBequivalent=0
  V_meas_bus : spsVoltageMeasurementLib/Voltage Measurement  PhasorSimulation=off  OutputType=Complex  PSBequivalent=0
  V_ref : Constant  Value=400
  Weather_15min : ZeroOrderHold  SampleTime=dt
  Weather_Scope : Scope  NumInputPorts=2
      settings: ActiveDisplayYMinimum=-116.6156432836914  ActiveDisplayYMaximum=1049.5407895532228  DataLoggingVariableName=wxdata
  ZOH_I : ZeroOrderHold  SampleTime=0.0001
  ZOH_V : ZeroOrderHold  SampleTime=0.0001
  DC_Bus+ : PMIOPort  Side=Right
  DC_Bus- : PMIOPort  Port=2  Side=Right
  m1 : Outport
  m2 : Outport  Port=2
  wires:
  V_meas_bus/1 -> V_err/2, PV_Scope/5
  P_PV/1 -> PV_Scope/3
  I_meas/1 -> P_PV/2, PV_Scope/2, ZOH_I/1
  T_cell/1 -> Weather_Scope/2, PV/2
  NOCT_heating/1 -> T_cell/1
  PI_CV/1 -> Sat_CV/1
  Gate/1 -> SW/1
  Hour_of_day/1 -> Weather_15min/1
  V_err/1 -> PI_CV/1
  Carrier/1 -> PWM/2
  ZOH_V/1 -> PandO/1(Vpv)
  PandO/1(D) -> Mode/3
  Clock/1 -> Hour_of_day/1
  V_ref/1 -> V_err/1
  ZOH_I/1 -> PandO/2(Ipv)
  Tamb_profile/1 -> T_cell/2
  Weather_15min/1 -> G_profile/1, Tamb_profile/1
  G_profile/1 -> PV/1, Weather_Scope/1, NOCT_heating/1
  SOC_full/1 -> Mode/2
  PWM/1 -> Gate/1
  V_meas_PV/1 -> ZOH_V/1, P_PV/1, PV_Scope/1
  Sat_CV/1 -> Mode/1
  Mode/1 -> PWM/1, PV_Scope/4
  SW/1 -> m2/1
  PV/1 -> m1/1
  [SoC_Battery] -> SOC_full/1
  connections:
  C_out/LConn1 -- V_meas_bus/LConn1 -- DC_Bus+/RConn1 -- D/RConn1
  C_in/RConn1 -- SW/RConn1 -- C_out/RConn1 -- PV/RConn2 -- V_meas_PV/LConn2 -- V_meas_bus/LConn2 -- DC_Bus-/RConn1
  C_in/LConn1 -- V_meas_PV/LConn1 -- I_meas/RConn1 -- L/LConn1
  SW/LConn1 -- D/LConn1 -- L/RConn1
  PV/RConn1 -- I_meas/LConn1

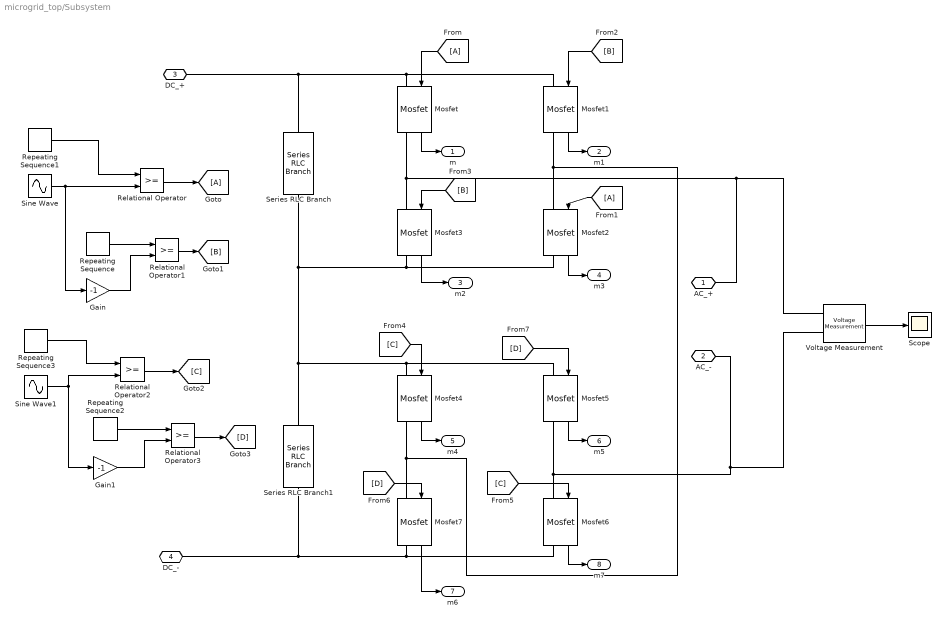
== system microgrid_top/Subsystem ==
  From : From
  From1 : From
  Gain : Gain  Gain=-1
  Gain1 : Gain  Gain=-1
  Goto : Goto
  Mosfet{,1..7} (8 alike) : spsMosfetLib/Mosfet  Ron=0.1  Lon=0  Rd=0.01  Vfd=0  IC=0  Rs=1e5  Cs=inf  Measurements=on
  Relational Operator{,1..3} (4 alike) : RelationalOperator  OutDataTypeStr=boolean  RndMeth=Simplest  InputSameDT=off
  Repeating Sequence : simulink/Sources/Repeating Sequence  rep_seq_t=[0 1]  rep_seq_y=[0 1]
  Repeating Sequence1 : simulink/Sources/Repeating Sequence  rep_seq_t=[0 1]  rep_seq_y=[0 1]
  Repeating Sequence2 : simulink/Sources/Repeating Sequence  rep_seq_t=[0 1]  rep_seq_y=[1 2]
  Repeating Sequence3 : simulink/Sources/Repeating Sequence  rep_seq_t=[0 1]  rep_seq_y=[1 2]
  Scope : Scope
      settings: ActiveDisplayYMinimum=-124.50174  ActiveDisplayYMaximum=124.50174
  Series RLC Branch : spsSeriesRLCBranchLib/Series RLC Branch  LConnTagsString=__new0  RConnTagsString=__new0  BranchType=C  Resistance=1  Inductance=1e-3  SetiL0=off  InitialCurrent=0  Capacitance=2200e-6  Setx0=off  InitialVoltage=0  Measurements=None
  Series RLC Branch1 : spsSeriesRLCBranchLib/Series RLC Branch  LConnTagsString=__new0  RConnTagsString=__new0  BranchType=C  Resistance=1  Inductance=1e-3  SetiL0=off  InitialCurrent=0  Capacitance=2200e-6  Setx0=off  InitialVoltage=0  Measurements=None
  Sine Wave : Sin  Amplitude=2  Frequency=2*pi*60  SampleTime=0
  Sine Wave1 : Sin  Amplitude=2  Frequency=2*pi*60  SampleTime=0
  Voltage Measurement : spsVoltageMeasurementLib/Voltage Measurement  PhasorSimulation=off  OutputType=Complex  PSBequivalent=0
  AC_+ : PMIOPort  Side=Right
  AC_- : PMIOPort  Port=2  Side=Right
  DC_+ : PMIOPort  Port=3  Side=Left
  DC_- : PMIOPort  Port=4  Side=Left
  m : Outport
  m1 : Outport  Port=2
  m2 : Outport  Port=3
  m3 : Outport  Port=4
  m4 : Outport  Port=5
  m5 : Outport  Port=6
  m6 : Outport  Port=7
  m7 : Outport  Port=8
  wires:
  Gain/1 -> Relational Operator1/2
  Mosfet5/1 -> m5/1
  Relational Operator1/1 -> [B]
  Mosfet4/1 -> m4/1
  Sine Wave/1 -> Relational Operator/2, Gain/1
  [B] -> Mosfet3/1
  Repeating Sequence1/1 -> Relational Operator/1
  Relational Operator2/1 -> [C]
  [B] -> Mosfet1/1
  Voltage Measurement/1 -> Scope/1
  From1/1 -> Mosfet2/1
  Mosfet7/1 -> m6/1
  Repeating Sequence2/1 -> Relational Operator3/1
  Sine Wave1/1 -> Relational Operator2/2, Gain1/1
  Relational Operator3/1 -> [D]
  Repeating Sequence/1 -> Relational Operator1/1
  [C] -> Mosfet4/1
  [D] -> Mosfet5/1
  Gain1/1 -> Relational Operator3/2
  Mosfet1/1 -> m1/1
  From/1 -> Mosfet/1
  [D] -> Mosfet7/1
  [C] -> Mosfet6/1
  Repeating Sequence3/1 -> Relational Operator2/1
  Relational Operator/1 -> Goto/1
  Mosfet2/1 -> m3/1
  Mosfet3/1 -> m2/1
  Mosfet/1 -> m/1
  Mosfet6/1 -> m7/1
  connections:
  Mosfet3/RConn1 -- Mosfet2/RConn1 -- Series RLC Branch1/LConn1 -- Mosfet5/LConn1 -- Mosfet4/LConn1 -- Series RLC Branch/RConn1
  Mosfet/RConn1 -- Mosfet3/LConn1 -- Voltage Measurement/LConn1 -- AC_+/RConn1
  Mosfet5/RConn1 -- Mosfet6/LConn1 -- Voltage Measurement/LConn2 -- AC_-/RConn1
  Series RLC Branch1/RConn1 -- Mosfet7/RConn1 -- Mosfet6/RConn1 -- DC_-/RConn1
  Mosfet4/RConn1 -- Mosfet7/LConn1 -- Mosfet1/RConn1 -- Mosfet2/LConn1
  Series RLC Branch/LConn1 -- Mosfet1/LConn1 -- Mosfet/LConn1 -- DC_+/RConn1

== matlab function microgrid_top/Loads/MATLAB Function ==
  data: t input; Preq output; Pact output; L input; epsn input; Edef_out output; dt parameter; Pmax parameter; prof parameter; Tc parameter; Emax parameter; sig parameter
function [Preq, Pact, Edef_out] = loads_func(t, L, epsn, dt, Pmax, prof, Tc, Emax, sig)
% LOADS_FUNC Computes tier-wise requested and active load power based on 
% Stateflow shedding level L and updates deferred unserved energy.
%
% Inputs:
%   t     - Current simulation time [s]
%   L     - Shedding level from Stateflow (0 = Normal, 1 = Shed Group 3, 2 = Shed Group 2&3, 3 = Blackout)
%   epsn  - Load variability noise
%   dt    - Macro time step in hours (0.25 h)
%   Pmax  - Max capacity limit [kW]
%   prof  - Base load profile matrix [24x3] for 12 flats
%   Tc    - Time constant for recovery
%   Emax  - Max allowable deferred energy [kWh]
%   sig   - Scaling factor
%
% Outputs:
%   Preq     - Requested load power per tier [P1, P2, P3] in kW
%   Pact     - Actual connected load power per tier [P1, P2, P3] in kW
%   Edef_out - Cumulative unserved energy [kWh]

persistent Edef u_prev

if isempty(Edef)
    Edef = 0;
end

if isempty(u_prev)
    u_prev = [1; 1; 1]; % All loads enabled by default
end

% 1. Decode Stateflow Shedding Level L into Tier Enable Vector u = [u1, u2, u3]
switch L
    case 0
        u = [1; 1; 1]; % L0: Normal - Group 1, 2, 3 Active
    case 1
        u = [1; 1; 0]; % L1: Shed Deferrable - Group 3 Off
    case 2
        u = [1; 0; 0]; % L2: Critical Only - Group 2 & 3 Off
    case 3
        u = [0; 0; 0]; % L3: Blackout / Outage - All Loads Off
    otherwise
        u = [1; 1; 1];
end

% 2. Calculate Time-of-Day Index (0 - 23 hours)
tod_hour = floor(mod(t / 3600, 24)) + 1; % 1-based indexing for MATLAB

% 3. Extract Baseline Power per Tier from 12-Flat Profile
% Tier 1 (Critical): Fridges, Routers, Emergency Lighting (~1.80 kW)
% Tier 2 (Essential): Lighting, Fans, TVs (~4.21 kW)
% Tier 3 (Deferrable): ACs, Geysers, Water Pumps (~18.75 kW)
P1_base = prof(tod_hour, 1);
P2_base = prof(tod_hour, 2);
P3_base = prof(tod_hour, 3);

% 4. Apply Variability Noise
Preq = [P1_base; P2_base; P3_base] .* (1 + epsn);

% 5. Compute Actual Connected Power
Pact = Preq .* u;

% 6. Track Unserved Deferrable Energy (Accumulated when Group 3 is shed)
P3_unserved = Preq(3) * (1 - u(3)); % kW of shed deferrable load
Edef = Edef + P3_unserved * dt;     % kW * hours = kWh

% If load is re-enabled, decay the deferred energy tracker
if u(3) == 1 && Edef > 0
    Edef = max(0, Edef - (Edef / Tc) * dt);
end

Edef = min(Edef, Emax); % Saturation limit
Edef_out = Edef;

u_prev = u;
end

== matlab function microgrid_top/BESS/MATLAB Function ==
  data: Pbat_base input; Pbat_adaptive output; SOC_Bat input
function Pbat_adaptive = fcn(Pbat_base, SOC_Bat)

if SOC_Bat < 30 && Pbat_base > 0
    Pbat_adaptive = 0.2 * Pbat_base;

elseif SOC_Bat > 90 && Pbat_base < 0
    Pbat_adaptive = 0.2 * Pbat_base;

else
    Pbat_adaptive = Pbat_base;
end

== stateflow chart microgrid_top/Load Manager ==
  settings: updateMethod=DISCRETE  sampleTime=0.25
  state L0_Normal
    en:L=0
    outage_flag = 0;
  state L1_ShedDeferrable
    en:L=1;
    outage_flag = 0;
  state L2_CriticalOnly
    en:L=2;
    outage_flag = 0;
  state L3_Outage
    en: L = 3;
    outage_flag = 1;
  L1_ShedDeferrable -> L2_CriticalOnly [order 1] : [SoC < th2_act]
  L0_Normal -> L1_ShedDeferrable : [SoC < th1_act || (SoC < th1_act + 0.05 && dSoC_dt < -0.15)]
  L2_CriticalOnly -> L3_Outage [order 2] : [SoC <= SoC_min || P_def > 22]
  (default) -> L0_Normal
  L3_Outage -> L0_Normal : [SoC > SoC_min + 0.10 && P_def <= 10]
  L1_ShedDeferrable -> L0_Normal [order 2] : [SoC>th1_act+d]
  L2_CriticalOnly -> L1_ShedDeferrable [order 1] : [SoC>th2_act+d]
  data: SoC input; L output; th1 parameter; th2 parameter; d parameter; dSoC_dt input; P_def input; SoC_min parameter; outage_flag output; th2_act parameter; th1_act parameter

== matlab function microgrid_top/PV Generation/PandO ==
  data: Vpv input; D output; Ipv input
function D = PandO(Vpv, Ipv)
% P&O MPPT with night parking, for a boost converter on a 400 V bus.
% Vpv = (1 - D) * Vbus, so lowering D raises the PV voltage.
persistent Vold Pold Dold
if isempty(Vold), Vold = 0; Pold = 0; Dold = 0.42; end
dD = 0.002;  Pmin = 50;  D_park = 0.42;
P  = Vpv*Ipv;  dV = Vpv - Vold;  dP = P - Pold;
if P < Pmin          % night or very weak light: park near 0.8*Voc
    D = D_park;
elseif dP == 0
    D = Dold;
elseif dP*dV > 0     % left of MPP: raise Vpv by lowering D
    D = Dold - dD;
else                 % right of MPP: lower Vpv by raising D
    D = Dold + dD;
end
% Voltage window: Vpv command 160-256 V (D 0.36-0.60). Covers every MPP
% of the day (~195-245 V) but never asks for more than Voc (~255+ V),
% so P&O cannot drift to open circuit when irradiance rises at sunrise.
D = min(max(D, 0.36), 0.60);
Vold = Vpv; Pold = P; Dold = D;
